simulink model "gm_uz_JL_flt_stop"  (R2025a)
settings: Solver=FixedStepDiscrete  StartTime=0.0  StopTime=inf  RelTol=1e-3
libraries: simulink_extras x6, hdlsllib x1
settings Model: Creator=jonat  LastModifiedBy=jonat
settings SolverCC: AlgebraicLoopSolver=TrustRegion
settings DataIOCC: LimitDataPoints=on  SaveOutput=off  SaveTime=off
settings OptimizationCC: BlockReduction=off  ConditionallyExecuteInputs=off  DefaultParameterBehavior=Inlined  InheritOutputTypeSmallerThanSingle=on  LifeSpan=inf
settings DebuggingCC: AlgebraicLoopMsg=error  InheritedTsInSrcMsg=none  SingleTaskRateTransMsg=error  UnconnectedInputMsg=warning  UnconnectedOutputMsg=warning  UnconnectedLineMsg=warning  AllowSymbolicDim=off  StrictBusMsg=ErrorOnBusTreatedAsVector  SFUnexpectedBacktrackingDiag=warning  SFNoUnconditionalDefaultTransitionDiag=warning  SFExecutionAtInitializationDiag=none  ArithmeticOperatorsInVariantConditions=warning
settings HardwareCC: ProdBitPerPointer=32.0  ProdBitPerSizeT=32.0  ProdBitPerPtrDiffT=32.0  ProdLargestAtomicFloat=None  ProdIntDivRoundTo=Undefined  ProdEndianess=Unspecified  ProdWordSize=32.0  ProdHWDeviceType=ASIC/FPGA->ASIC/FPGA  ProdEqTarget=off
settings ModelReferenceCC: EnableRefExpFcnMdlSchedulingChecks=on
settings SFSimCC: SimUseLocalCustomCode=off  CustomCodeUndefinedFunction=UseInterfaceOnly
settings RTWCC: RTWUseLocalCustomCode=off  GPUComputeCapability=3.5
settings CodeAppCC: StateflowObjectComments=on
settings GRTTargetCC: TargetLangStandard=C89/C90 (ANSI)
settings ConfigComp: CovScope=ReferencedModels  CovMetricSettings=dw  CovSaveCumulativeToWorkspaceVar=on  CovSaveSingleToWorkspaceVar=on  CovExternalEMLEnable=off  CovSFcnEnable=off

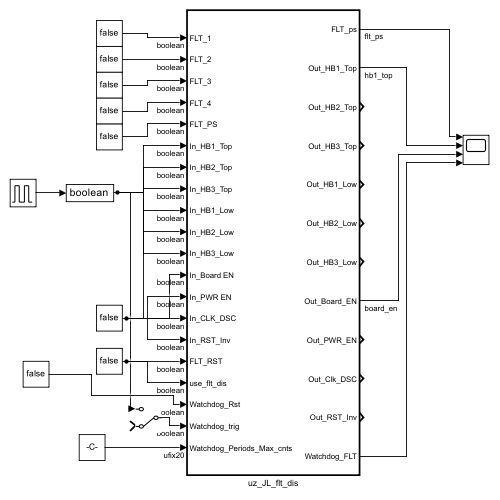
[thumbnail: Simulink's stored preview of the top-level diagram]
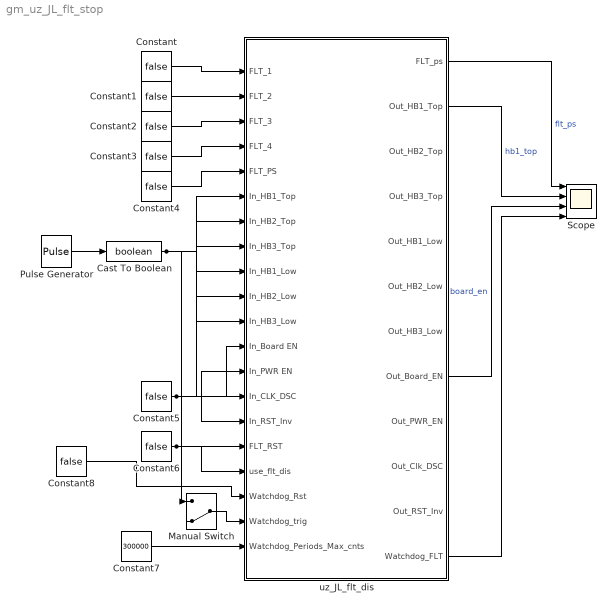
== system gm_uz_JL_flt_stop ==
  Cast To Boolean : DataTypeConversion  OutDataTypeStr=boolean  SaturateOnIntegerOverflow=off  RndMeth=Floor
  Constant{,1..6,8} (8 alike) : Constant  Value=false  OutDataTypeStr=boolean
  Constant7 : Constant  Value=300000  OutDataTypeStr=fixdt(0,20,0)
  Manual Switch : ManualSwitch  CurrentSetting=0
  Pulse Generator : DiscretePulseGenerator  PulseType=Time based  Period=1/10e3  PulseWidth=50
  Scope : Scope  NumInputPorts=4
      settings: ActiveDisplayYMinimum=-0.12499999999999997  ActiveDisplayYMaximum=1.125
  uz_JL_flt_dis : Subsystem  TreatAsAtomicUnit=on
  wires:
  Constant8/1 -> uz_JL_flt_dis/18(Watchdog_Rst)
  Manual Switch/1 -> uz_JL_flt_dis/19(Watchdog_trig)
  uz_JL_flt_dis/12(Watchdog_FLT) -> Scope/4
  Constant7/1 -> uz_JL_flt_dis/20(Watchdog_Periods_Max_cnts)
  Cast To Boolean/1 -> uz_JL_flt_dis/9(In_HB1_Low), uz_JL_flt_dis/10(In_HB2_Low), uz_JL_flt_dis/11(In_HB3_Low), uz_JL_flt_dis/14(In_CLK_DSC), uz_JL_flt_dis/7(In_HB2_Top), uz_JL_flt_dis/6(In_HB1_Top), uz_JL_flt_dis/8(In_HB3_Top), Manual Switch/1
  uz_JL_flt_dis/8(Out_Board_EN) -> Scope/3  "board_en"
  uz_JL_flt_dis/2(Out_HB1_Top) -> Scope/2  "hb1_top"
  uz_JL_flt_dis/1(FLT_ps) -> Scope/1  "flt_ps"
  Constant6/1 -> uz_JL_flt_dis/16(FLT_RST), uz_JL_flt_dis/17(use_flt_dis)
  Constant5/1 -> uz_JL_flt_dis/12(In_Board EN), uz_JL_flt_dis/13(In_PWR EN), uz_JL_flt_dis/15(In_RST_Inv)
  Pulse Generator/1 -> Cast To Boolean/1
  Constant4/1 -> uz_JL_flt_dis/5(FLT_PS)
  Constant3/1 -> uz_JL_flt_dis/4(FLT_4)
  Constant2/1 -> uz_JL_flt_dis/3(FLT_3)
  Constant1/1 -> uz_JL_flt_dis/2(FLT_2)
  Constant/1 -> uz_JL_flt_dis/1(FLT_1)

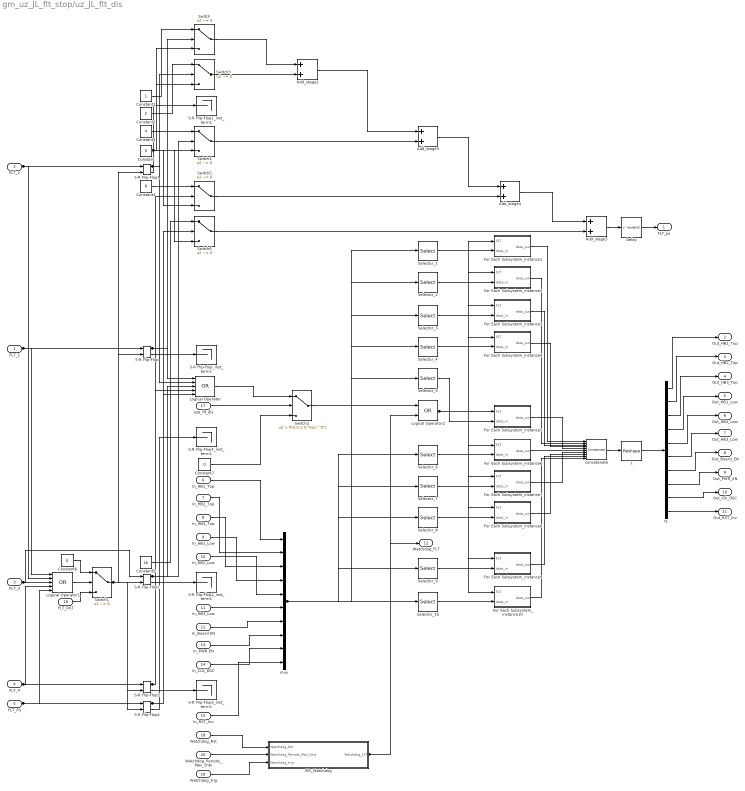
== system gm_uz_JL_flt_stop/uz_JL_flt_dis ==
  FLT_1 : Inport  OutDataTypeStr=boolean  PortDimensions=1  SampleTime=5e-05
  FLT_2 : Inport  Port=2  OutDataTypeStr=boolean  PortDimensions=1  SampleTime=5e-05
  FLT_3 : Inport  Port=3  OutDataTypeStr=boolean  PortDimensions=1  SampleTime=5e-05
  FLT_4 : Inport  Port=4  OutDataTypeStr=boolean  PortDimensions=1  SampleTime=5e-05
  FLT_PS : Inport  Port=5  OutDataTypeStr=boolean  PortDimensions=1  SampleTime=5e-05
  In_HB1_Top : Inport  Port=6  OutDataTypeStr=boolean  PortDimensions=1  SampleTime=5e-05
  In_HB2_Top : Inport  Port=7  OutDataTypeStr=boolean  PortDimensions=1  SampleTime=5e-05
  In_HB3_Top : Inport  Port=8  OutDataTypeStr=boolean  PortDimensions=1  SampleTime=5e-05
  In_HB1_Low : Inport  Port=9  OutDataTypeStr=boolean  PortDimensions=1  SampleTime=5e-05
  In_HB2_Low : Inport  Port=10  OutDataTypeStr=boolean  PortDimensions=1  SampleTime=5e-05
  In_HB3_Low : Inport  Port=11  OutDataTypeStr=boolean  PortDimensions=1  SampleTime=5e-05
  In_Board EN : Inport  Port=12  OutDataTypeStr=boolean  PortDimensions=1  SampleTime=5e-05
  In_PWR EN : Inport  Port=13  OutDataTypeStr=boolean  PortDimensions=1  SampleTime=5e-05
  In_CLK_DSC : Inport  Port=14  OutDataTypeStr=boolean  PortDimensions=1  SampleTime=5e-05
  In_RST_Inv : Inport  Port=15  OutDataTypeStr=boolean  PortDimensions=1  SampleTime=5e-05
  FLT_RST : Inport  Port=16  OutDataTypeStr=boolean  PortDimensions=1  SampleTime=5e-05
  use_flt_dis : Inport  Port=17  OutDataTypeStr=boolean  PortDimensions=1  SampleTime=5e-05
  Watchdog_Rst : Inport  Port=18  OutDataTypeStr=boolean  PortDimensions=1  SampleTime=5e-05
  Watchdog_trig : Inport  Port=19  OutDataTypeStr=boolean  PortDimensions=1  SampleTime=5e-05
  Watchdog_Periods_Max_cnts : Inport  Port=20  OutDataTypeStr=fixdt(0, 20, 0)  PortDimensions=1  SampleTime=5e-05
  Add_stage2 : Sum  OutDataTypeStr=fixdt(0, 9, 0)  AccumDataTypeStr=fixdt(0, 11, 0)  SampleTime=5e-05
  Add_stage3 : Sum  OutDataTypeStr=fixdt(0, 10, 0)  AccumDataTypeStr=fixdt(0, 11, 0)  SampleTime=5e-05
  Add_stage4 : Sum  OutDataTypeStr=fixdt(0, 11, 0)  AccumDataTypeStr=fixdt(0, 11, 0)  SampleTime=5e-05
  Add_stage5 : Sum  OutDataTypeStr=fixdt(0, 11, 0)  AccumDataTypeStr=fixdt(0, 11, 0)  SampleTime=5e-05
  Constant : Constant  Value=0  OutDataTypeStr=uint8  SampleTime=5e-05
  Constant1 : Constant  OutDataTypeStr=uint8  SampleTime=5e-05
  Constant2 : Constant  Value=2  OutDataTypeStr=uint8  SampleTime=5e-05
  Constant3 : Constant  Value=4  OutDataTypeStr=uint8  SampleTime=5e-05
  Constant4 : Constant  Value=8  OutDataTypeStr=uint8  SampleTime=5e-05
  Constant5 : Constant  Value=16  OutDataTypeStr=uint8  SampleTime=5e-05
  Constant6 : Constant  Value=0  OutDataTypeStr=boolean  SampleTime=5e-05
  Constant7 : Constant  Value=0  OutDataTypeStr=boolean  SampleTime=5e-05
  Delay : Delay  DelayLength=double(1)  InitialCondition=0  SampleTime=5e-05
  For Each Subsystem_instance1 : Subsystem
  For Each Subsystem_instance10 : Subsystem
  For Each Subsystem_instance2 : Subsystem
  For Each Subsystem_instance3 : Subsystem
  For Each Subsystem_instance4 : Subsystem
  For Each Subsystem_instance5 : Subsystem
  For Each Subsystem_instance6 : Subsystem
  For Each Subsystem_instance7 : Subsystem
  For Each Subsystem_instance8 : Subsystem
  For Each Subsystem_instance9 : Subsystem
  ISR_Watchdog : Subsystem
  Logical Operator : Logic  Operator=OR  Inputs=5  AllPortsSameDT=off  OutDataTypeStr=boolean  SampleTime=5e-05
  Logical Operator1 : Logic  Operator=OR  Inputs=5  AllPortsSameDT=off  OutDataTypeStr=boolean  SampleTime=5e-05
  Logical Operator2 : Logic  Operator=OR  AllPortsSameDT=off  OutDataTypeStr=boolean  SampleTime=5e-05
  S-R Flip-Flop{,1..4} (5 alike) : simulink_extras/Flip Flops/S-R Flip-Flop  initial_condition=0
  S-R Flip-Flop1_inst_term1 : Terminator
  S-R Flip-Flop2_inst_term1 : Terminator
  S-R Flip-Flop3_inst_term1 : Terminator
  S-R Flip-Flop4_inst_term1 : Terminator
  S-R Flip-Flop_inst_term1 : Terminator
  Selector_1 : Selector  InputPortWidth=10  IndexOptions=Index vector (dialog)  Indices=double(1)  OutputSizes=1
  Selector_10 : Selector  InputPortWidth=10  IndexOptions=Index vector (dialog)  Indices=double(10)  OutputSizes=1
  Selector_2 : Selector  InputPortWidth=10  IndexOptions=Index vector (dialog)  Indices=double(2)  OutputSizes=1
  Selector_3 : Selector  InputPortWidth=10  IndexOptions=Index vector (dialog)  Indices=double(3)  OutputSizes=1
  Selector_4 : Selector  InputPortWidth=10  IndexOptions=Index vector (dialog)  Indices=double(4)  OutputSizes=1
  Selector_5 : Selector  InputPortWidth=10  IndexOptions=Index vector (dialog)  Indices=double(5)  OutputSizes=1
  Selector_6 : Selector  InputPortWidth=10  IndexOptions=Index vector (dialog)  Indices=double(6)  OutputSizes=1
  Selector_7 : Selector  InputPortWidth=10  IndexOptions=Index vector (dialog)  Indices=double(7)  OutputSizes=1
  Selector_8 : Selector  InputPortWidth=10  IndexOptions=Index vector (dialog)  Indices=double(8)  OutputSizes=1
  Selector_9 : Selector  InputPortWidth=10  IndexOptions=Index vector (dialog)  Indices=double(9)  OutputSizes=1
  Switch{,3..6} (5 alike) : Switch  Criteria=u2 ~= 0  Threshold="fi(0,0,1,0,\"hex\",\"0\")"  OutDataTypeStr=uint8  SampleTime=5e-05  SaturateOnIntegerOverflow=off  InputSameDT=off
  Switch1 : Switch  Criteria=u2 ~= 0  Threshold="fi(0,0,1,0,\"hex\",\"0\")"  OutDataTypeStr=boolean  SampleTime=5e-05  SaturateOnIntegerOverflow=off  InputSameDT=off
  Switch2 : Switch  Criteria=u2 > Threshold  Threshold="fi(0,0,1,0,\"hex\",\"0\")"  OutDataTypeStr=boolean  SampleTime=5e-05  SaturateOnIntegerOverflow=off  InputSameDT=off
  concatenate : Concatenate  NumInputs=10
  mux : Mux  Inputs=10
  t : Reshape
  t1 : Demux  Outputs=10
  FLT_ps : Outport  SampleTime=5e-05
  Out_HB1_Top : Outport  Port=2  SampleTime=5e-05
  Out_HB2_Top : Outport  Port=3  SampleTime=5e-05
  Out_HB3_Top : Outport  Port=4  SampleTime=5e-05
  Out_HB1_Low : Outport  Port=5  SampleTime=5e-05
  Out_HB2_Low : Outport  Port=6  SampleTime=5e-05
  Out_HB3_Low : Outport  Port=7  SampleTime=5e-05
  Out_Board_EN : Outport  Port=8  SampleTime=5e-05
  Out_PWR_EN : Outport  Port=9  SampleTime=5e-05
  Out_Clk_DSC : Outport  Port=10  SampleTime=5e-05
  Out_RST_Inv : Outport  Port=11  SampleTime=5e-05
  Watchdog_FLT : Outport  Port=12  SampleTime=5e-05
  wires:
  FLT_2/1 -> S-R Flip-Flop1/1, Logical Operator1/2
  Selector_9/1 -> For Each Subsystem_instance9/2(data_in)
  Constant6/1 -> Switch1/1
  FLT_RST/1 -> Switch1/3
  FLT_PS/1 -> S-R Flip-Flop4/1, Logical Operator1/5
  FLT_1/1 -> S-R Flip-Flop/1, Logical Operator1/1
  Constant2/1 -> Switch3/1
  FLT_3/1 -> S-R Flip-Flop2/1, Logical Operator1/3
  Logical Operator1/1 -> Switch1/2
  FLT_4/1 -> S-R Flip-Flop3/1, Logical Operator1/4
  In_HB2_Low/1 -> mux/5
  Switch1/1 -> S-R Flip-Flop4/2, S-R Flip-Flop1/2, S-R Flip-Flop2/2, S-R Flip-Flop/2, S-R Flip-Flop3/2
  Constant1/1 -> Switch/1
  Selector_7/1 -> For Each Subsystem_instance7/2(data_in)
  Constant3/1 -> Switch4/1
  Selector_5/1 -> For Each Subsystem_instance5/2(data_in)
  Constant/1 -> Switch4/3, Switch3/3, Switch6/3, Switch/3, Switch5/3
  S-R Flip-Flop1/1 -> Switch3/2, Logical Operator/2
  S-R Flip-Flop1/2 -> S-R Flip-Flop1_inst_term1/1
  Constant4/1 -> Switch5/1
  t1/4 -> Out_HB1_Low/1
  In_HB1_Top/1 -> mux/1
  S-R Flip-Flop/1 -> Switch/2, Logical Operator/1
  S-R Flip-Flop/2 -> S-R Flip-Flop_inst_term1/1
  Constant5/1 -> Switch6/1
  S-R Flip-Flop2/1 -> Switch4/2, Logical Operator/3
  Selector_8/1 -> For Each Subsystem_instance8/2(data_in)
  S-R Flip-Flop2/2 -> S-R Flip-Flop2_inst_term1/1
  Add_stage2/1 -> Add_stage3/1
  S-R Flip-Flop3/1 -> Switch5/2, Logical Operator/4
  Selector_1/1 -> For Each Subsystem_instance1/2(data_in)
  S-R Flip-Flop3/2 -> S-R Flip-Flop3_inst_term1/1
  Switch/1 -> Add_stage2/1
  S-R Flip-Flop4/1 -> Switch6/2, Logical Operator/5
  S-R Flip-Flop4/2 -> S-R Flip-Flop4_inst_term1/1
  Logical Operator2/1 -> For Each Subsystem_instance10/1(FLT), For Each Subsystem_instance9/1(FLT), For Each Subsystem_instance8/1(FLT), For Each Subsystem_instance6/1(FLT), For Each Subsystem_instance5/1(FLT), For Each Subsystem_instance7/1(FLT), For Each Subsystem_instance4/1(FLT), For Each Subsystem_instance2/1(FLT), For Each Subsystem_instance3/1(FLT), For Each Subsystem_instance1/1(FLT)
  Watchdog_trig/1 -> ISR_Watchdog/3(Watchdog_trig)
  Switch3/1 -> Add_stage2/2
  Switch4/1 -> Add_stage3/2
  t1/6 -> Out_HB3_Low/1
  In_RST_Inv/1 -> mux/10
  Switch5/1 -> Add_stage4/2
  Switch6/1 -> Add_stage5/2
  Logical Operator/1 -> Switch2/1
  use_flt_dis/1 -> Switch2/2
  Constant7/1 -> Switch2/3
  For Each Subsystem_instance1/1(data_out) -> concatenate/1
  In_HB2_Top/1 -> mux/2
  In_HB3_Top/1 -> mux/3
  Add_stage5/1 -> Delay/1
  In_HB1_Low/1 -> mux/4
  In_HB3_Low/1 -> mux/6
  In_Board EN/1 -> mux/7
  Selector_6/1 -> For Each Subsystem_instance6/2(data_in)
  In_PWR EN/1 -> mux/8
  t1/10 -> Out_RST_Inv/1
  In_CLK_DSC/1 -> mux/9
  Watchdog_Rst/1 -> ISR_Watchdog/1(Watchdog_Rst)
  Selector_2/1 -> For Each Subsystem_instance2/2(data_in)
  Watchdog_Periods_Max_cnts/1 -> ISR_Watchdog/2(Watchdog_Periods_Max_Cnts)
  Switch2/1 -> Logical Operator2/1
  mux/1 -> Selector_10/1, Selector_9/1, Selector_8/1, Selector_7/1, Selector_6/1, Selector_3/1, Selector_1/1, Selector_2/1, Selector_4/1, Selector_5/1
  ISR_Watchdog/1(Watchdog_FLT) -> Logical Operator2/2, Watchdog_FLT/1
  Add_stage3/1 -> Add_stage4/1
  Selector_3/1 -> For Each Subsystem_instance3/2(data_in)
  Selector_4/1 -> For Each Subsystem_instance4/2(data_in)
  Selector_10/1 -> For Each Subsystem_instance10/2(data_in)
  Add_stage4/1 -> Add_stage5/1
  For Each Subsystem_instance2/1(data_out) -> concatenate/2
  For Each Subsystem_instance3/1(data_out) -> concatenate/3
  For Each Subsystem_instance4/1(data_out) -> concatenate/4
  For Each Subsystem_instance5/1(data_out) -> concatenate/5
  For Each Subsystem_instance6/1(data_out) -> concatenate/6
  For Each Subsystem_instance7/1(data_out) -> concatenate/7
  For Each Subsystem_instance8/1(data_out) -> concatenate/8
  For Each Subsystem_instance9/1(data_out) -> concatenate/9
  For Each Subsystem_instance10/1(data_out) -> concatenate/10
  concatenate/1 -> t/1
  Delay/1 -> FLT_ps/1
  t/1 -> t1/1
  t1/1 -> Out_HB1_Top/1
  t1/2 -> Out_HB2_Top/1
  t1/3 -> Out_HB3_Top/1
  t1/5 -> Out_HB2_Low/1
  t1/7 -> Out_Board_EN/1
  t1/8 -> Out_PWR_EN/1
  t1/9 -> Out_Clk_DSC/1

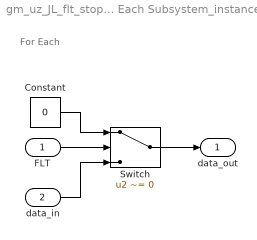
== system gm_uz_JL_flt_stop/uz_JL_flt_dis/For Each Subsystem_instance1 ==
  note: For Each
  FLT : Inport  OutDataTypeStr=boolean  PortDimensions=1  SampleTime=5e-05
  data_in : Inport  Port=2  OutDataTypeStr=boolean  PortDimensions=1  SampleTime=5e-05
  Constant : Constant  Value=0  OutDataTypeStr=boolean  SampleTime=-1
  Switch : Switch  Criteria=u2 ~= 0  OutDataTypeStr=boolean  SaturateOnIntegerOverflow=off  InputSameDT=off
  data_out : Outport  SampleTime=5e-05
  wires:
  data_in/1 -> Switch/3
  Constant/1 -> Switch/1
  FLT/1 -> Switch/2
  Switch/1 -> data_out/1

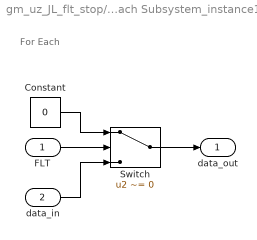
== system gm_uz_JL_flt_stop/uz_JL_flt_dis/For Each Subsystem_instance10 ==
  note: For Each
  FLT : Inport  OutDataTypeStr=boolean  PortDimensions=1  SampleTime=5e-05
  data_in : Inport  Port=2  OutDataTypeStr=boolean  PortDimensions=1  SampleTime=5e-05
  Constant : Constant  Value=0  OutDataTypeStr=boolean  SampleTime=-1
  Switch : Switch  Criteria=u2 ~= 0  OutDataTypeStr=boolean  SaturateOnIntegerOverflow=off  InputSameDT=off
  data_out : Outport  SampleTime=5e-05
  wires:
  Switch/1 -> data_out/1
  data_in/1 -> Switch/3
  Constant/1 -> Switch/1
  FLT/1 -> Switch/2

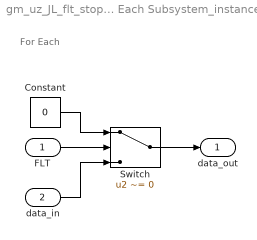
== system gm_uz_JL_flt_stop/uz_JL_flt_dis/For Each Subsystem_instance2 ==
  note: For Each
  FLT : Inport  OutDataTypeStr=boolean  PortDimensions=1  SampleTime=5e-05
  data_in : Inport  Port=2  OutDataTypeStr=boolean  PortDimensions=1  SampleTime=5e-05
  Constant : Constant  Value=0  OutDataTypeStr=boolean  SampleTime=-1
  Switch : Switch  Criteria=u2 ~= 0  OutDataTypeStr=boolean  SaturateOnIntegerOverflow=off  InputSameDT=off
  data_out : Outport  SampleTime=5e-05
  wires:
  Switch/1 -> data_out/1
  data_in/1 -> Switch/3
  Constant/1 -> Switch/1
  FLT/1 -> Switch/2

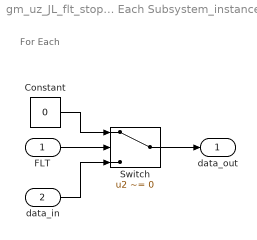
== system gm_uz_JL_flt_stop/uz_JL_flt_dis/For Each Subsystem_instance3 ==
  note: For Each
  FLT : Inport  OutDataTypeStr=boolean  PortDimensions=1  SampleTime=5e-05
  data_in : Inport  Port=2  OutDataTypeStr=boolean  PortDimensions=1  SampleTime=5e-05
  Constant : Constant  Value=0  OutDataTypeStr=boolean  SampleTime=-1
  Switch : Switch  Criteria=u2 ~= 0  OutDataTypeStr=boolean  SaturateOnIntegerOverflow=off  InputSameDT=off
  data_out : Outport  SampleTime=5e-05
  wires:
  Switch/1 -> data_out/1
  data_in/1 -> Switch/3
  Constant/1 -> Switch/1
  FLT/1 -> Switch/2

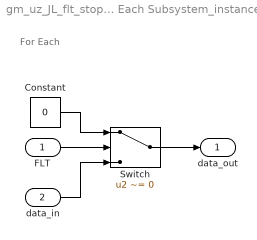
== system gm_uz_JL_flt_stop/uz_JL_flt_dis/For Each Subsystem_instance4 ==
  note: For Each
  FLT : Inport  OutDataTypeStr=boolean  PortDimensions=1  SampleTime=5e-05
  data_in : Inport  Port=2  OutDataTypeStr=boolean  PortDimensions=1  SampleTime=5e-05
  Constant : Constant  Value=0  OutDataTypeStr=boolean  SampleTime=-1
  Switch : Switch  Criteria=u2 ~= 0  OutDataTypeStr=boolean  SaturateOnIntegerOverflow=off  InputSameDT=off
  data_out : Outport  SampleTime=5e-05
  wires:
  Switch/1 -> data_out/1
  data_in/1 -> Switch/3
  Constant/1 -> Switch/1
  FLT/1 -> Switch/2

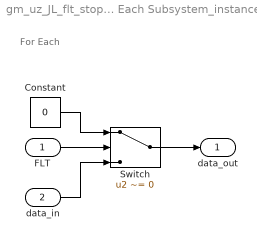
== system gm_uz_JL_flt_stop/uz_JL_flt_dis/For Each Subsystem_instance5 ==
  note: For Each
  FLT : Inport  OutDataTypeStr=boolean  PortDimensions=1  SampleTime=5e-05
  data_in : Inport  Port=2  OutDataTypeStr=boolean  PortDimensions=1  SampleTime=5e-05
  Constant : Constant  Value=0  OutDataTypeStr=boolean  SampleTime=-1
  Switch : Switch  Criteria=u2 ~= 0  OutDataTypeStr=boolean  SaturateOnIntegerOverflow=off  InputSameDT=off
  data_out : Outport  SampleTime=5e-05
  wires:
  FLT/1 -> Switch/2
  Constant/1 -> Switch/1
  data_in/1 -> Switch/3
  Switch/1 -> data_out/1

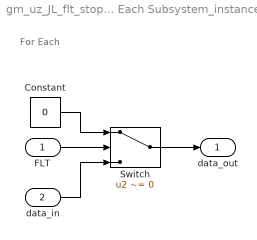
== system gm_uz_JL_flt_stop/uz_JL_flt_dis/For Each Subsystem_instance6 ==
  note: For Each
  FLT : Inport  OutDataTypeStr=boolean  PortDimensions=1  SampleTime=5e-05
  data_in : Inport  Port=2  OutDataTypeStr=boolean  PortDimensions=1  SampleTime=5e-05
  Constant : Constant  Value=0  OutDataTypeStr=boolean  SampleTime=-1
  Switch : Switch  Criteria=u2 ~= 0  OutDataTypeStr=boolean  SaturateOnIntegerOverflow=off  InputSameDT=off
  data_out : Outport  SampleTime=5e-05
  wires:
  Switch/1 -> data_out/1
  data_in/1 -> Switch/3
  Constant/1 -> Switch/1
  FLT/1 -> Switch/2

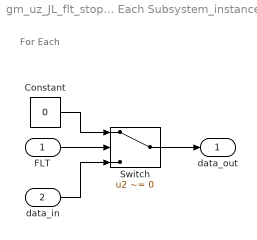
== system gm_uz_JL_flt_stop/uz_JL_flt_dis/For Each Subsystem_instance7 ==
  note: For Each
  FLT : Inport  OutDataTypeStr=boolean  PortDimensions=1  SampleTime=5e-05
  data_in : Inport  Port=2  OutDataTypeStr=boolean  PortDimensions=1  SampleTime=5e-05
  Constant : Constant  Value=0  OutDataTypeStr=boolean  SampleTime=-1
  Switch : Switch  Criteria=u2 ~= 0  OutDataTypeStr=boolean  SaturateOnIntegerOverflow=off  InputSameDT=off
  data_out : Outport  SampleTime=5e-05
  wires:
  Switch/1 -> data_out/1
  data_in/1 -> Switch/3
  Constant/1 -> Switch/1
  FLT/1 -> Switch/2

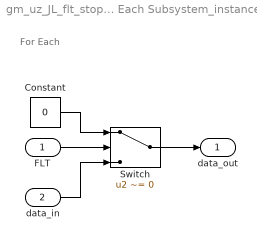
== system gm_uz_JL_flt_stop/uz_JL_flt_dis/For Each Subsystem_instance8 ==
  note: For Each
  FLT : Inport  OutDataTypeStr=boolean  PortDimensions=1  SampleTime=5e-05
  data_in : Inport  Port=2  OutDataTypeStr=boolean  PortDimensions=1  SampleTime=5e-05
  Constant : Constant  Value=0  OutDataTypeStr=boolean  SampleTime=-1
  Switch : Switch  Criteria=u2 ~= 0  OutDataTypeStr=boolean  SaturateOnIntegerOverflow=off  InputSameDT=off
  data_out : Outport  SampleTime=5e-05
  wires:
  data_in/1 -> Switch/3
  Constant/1 -> Switch/1
  FLT/1 -> Switch/2
  Switch/1 -> data_out/1

== system gm_uz_JL_flt_stop/uz_JL_flt_dis/For Each Subsystem_instance9 ==
  note: For Each
  FLT : Inport  OutDataTypeStr=boolean  PortDimensions=1  SampleTime=5e-05
  data_in : Inport  Port=2  OutDataTypeStr=boolean  PortDimensions=1  SampleTime=5e-05
  Constant : Constant  Value=0  OutDataTypeStr=boolean  SampleTime=-1
  Switch : Switch  Criteria=u2 ~= 0  OutDataTypeStr=boolean  SaturateOnIntegerOverflow=off  InputSameDT=off
  data_out : Outport  SampleTime=5e-05
  wires:
  Switch/1 -> data_out/1
  data_in/1 -> Switch/3
  Constant/1 -> Switch/1
  FLT/1 -> Switch/2

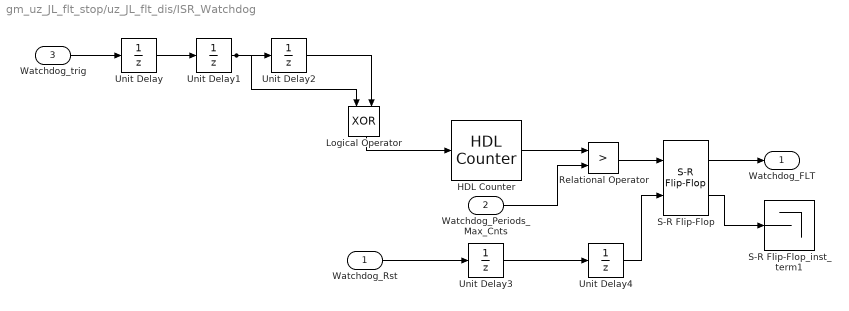
== system gm_uz_JL_flt_stop/uz_JL_flt_dis/ISR_Watchdog ==
  Watchdog_Rst : Inport  OutDataTypeStr=boolean  PortDimensions=1  SampleTime=5e-05
  Watchdog_Periods_Max_Cnts : Inport  Port=2  OutDataTypeStr=fixdt(0, 20, 0)  PortDimensions=1  SampleTime=5e-05
  Watchdog_trig : Inport  Port=3  OutDataTypeStr=boolean  PortDimensions=1  SampleTime=5e-05
  HDL Counter : hdlsllib/Sources/HDL Counter  CountType=Count limited  CountInit=1  CountStep=1  CountMax=1048575  CountFromType=Initial value  CountFrom=1  CountResetPort=on  CountLoadPort=off  CountEnbPort=off  CountDirPort=off  CountHitOutputPort=off  CountDataType=Unsigned  CountWordLen=20  CountFracLen=0  CountSampTime=1
  Logical Operator : Logic  Operator=XOR  AllPortsSameDT=off  OutDataTypeStr=boolean
  Relational Operator : RelationalOperator  Operator=>  OutDataTypeStr=boolean  RndMeth=Simplest  InputSameDT=off
  S-R Flip-Flop : simulink_extras/Flip Flops/S-R Flip-Flop  initial_condition=0
  S-R Flip-Flop_inst_term1 : Terminator
  Unit Delay{,1..4} (5 alike) : UnitDelay  SampleTime=-1  HasFrameUpgradeWarning=on
  Watchdog_FLT : Outport  SampleTime=5e-05
  wires:
  Unit Delay3/1 -> Unit Delay4/1
  Unit Delay1/1 -> Logical Operator/1, Unit Delay2/1
  Unit Delay/1 -> Unit Delay1/1
  Watchdog_trig/1 -> Unit Delay/1
  Watchdog_Periods_Max_Cnts/1 -> Relational Operator/2
  Unit Delay2/1 -> Logical Operator/2
  Logical Operator/1 -> HDL Counter/1
  Watchdog_Rst/1 -> Unit Delay3/1
  HDL Counter/1 -> Relational Operator/1
  Relational Operator/1 -> S-R Flip-Flop/1
  Unit Delay4/1 -> S-R Flip-Flop/2
  S-R Flip-Flop/1 -> Watchdog_FLT/1
  S-R Flip-Flop/2 -> S-R Flip-Flop_inst_term1/1
